simulink model "Controlador_PI"  (R2026b)
settings: Solver=ode4  FixedStep=0.1
InitFcn:
  | Kp = 1.1;
  | Ki = 1.83;
undefined symbols (not defined in the file): DiscIntNeverNeededParam, dspblkCoreblockFVToolHelper, gcbh
settings Model: Creator=joaov  LastModifiedBy=João
settings DataIOCC: ReturnWorkspaceOutputs=off
settings ConfigComp: PLC_Enable64bitIntSupport=off  PLC_EnableStringLiteralTB=on  PLC_EnableUDTSplitting=off  PLC_EnableUnsignedAndDoubleTypes=off  PLC_FoldFBCallOutputVar=off  PLC_InlineEnumCastFunction=off  PLC_MultiTBSigbuilderTimeRange=off  PLC_RemoveUnusedSSMethodCallArguments=off  PLC_TargetIDE=plcopen  PLC_UseCallOutputArgSyntax=off

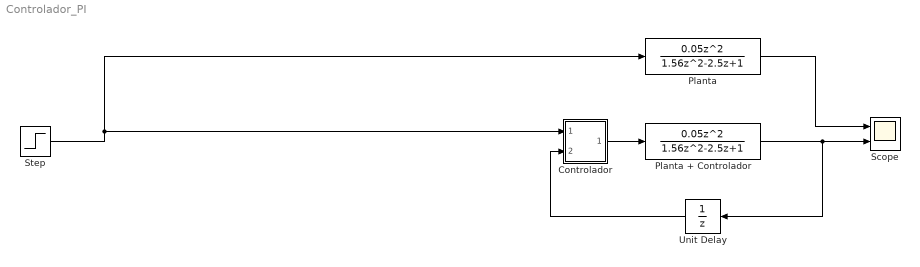
== system Controlador_PI ==
  Controlador : Subsystem  TreatAsAtomicUnit=on
  Planta : DiscreteTransferFcn  LoadFcn=dspblkCoreblockFVToolHelper(gcbh,'load');  Numerator=[0.05 0 0]  Denominator=[1.56 -2.5 1]
      settings: CopyFcn=dspblkCoreblockFVToolHelper(gcbh,'copy');  DeleteFcn=dspblkCoreblockFVToolHelper(gcbh,'close');  ModelCloseFcn=dspblkCoreblockFVToolHelper(gcbh,'close');  PreSaveFcn=dspblkCoreblockFVToolHelper(gcbh,'presave');  PostSaveFcn=dspblkCoreblockFVToolHelper(gcbh,'postsave');  CloseFcn=dspblkCoreblockFVToolHelper(gcbh,'close');
  Planta + Controlador : DiscreteTransferFcn  LoadFcn=dspblkCoreblockFVToolHelper(gcbh,'load');  Numerator=[0.05 0 0]  Denominator=[1.56 -2.5 1]
      settings: CopyFcn=dspblkCoreblockFVToolHelper(gcbh,'copy');  DeleteFcn=dspblkCoreblockFVToolHelper(gcbh,'close');  ModelCloseFcn=dspblkCoreblockFVToolHelper(gcbh,'close');  PreSaveFcn=dspblkCoreblockFVToolHelper(gcbh,'presave');  PostSaveFcn=dspblkCoreblockFVToolHelper(gcbh,'postsave');  CloseFcn=dspblkCoreblockFVToolHelper(gcbh,'close');
  Scope : Scope  NumInputPorts=2
      settings: ActiveDisplayYMinimum=-6.6606720028398287  ActiveDisplayYMaximum=77.814693561448252  DataLoggingVariableName=dados_subsistema
  Step : Step  FinalValue=50  SampleTime=0.1
  Unit Delay : UnitDelay  SampleTime=0.1
  wires:
  Planta + Controlador/1 -> Unit Delay/1, Scope/2
  Step/1 -> Controlador/1(In1), Planta/1
  Planta/1 -> Scope/1
  Unit Delay/1 -> Controlador/2(In2)
  Controlador/1(Out1) -> Planta + Controlador/1

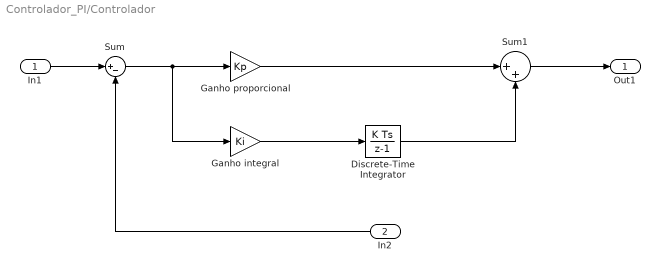
== system Controlador_PI/Controlador ==
  In1 : Inport
  In2 : Inport  Port=2
  Discrete-Time Integrator : DiscreteIntegrator  SampleTime=0.1  ICPrevOutput=DiscIntNeverNeededParam  ICPrevScaledInput=DiscIntNeverNeededParam
  Ganho integral : Gain  Gain=Ki
  Ganho proporcional : Gain  Gain=Kp
  Sum : Sum  Inputs=|+-
  Sum1 : Sum  Inputs=|++
  Out1 : Outport
  wires:
  Ganho integral/1 -> Discrete-Time Integrator/1
  In1/1 -> Sum/1
  Sum/1 -> Ganho integral/1, Ganho proporcional/1
  Sum1/1 -> Out1/1
  Ganho proporcional/1 -> Sum1/1
  Discrete-Time Integrator/1 -> Sum1/2
  In2/1 -> Sum/2
